simulink model "VoltageSourceConverterHVDCTrans"  (R2025b)
settings: Solver=FixedStepDiscrete  StartTime=0.0  StopTime=5  FixedStep=Ts  MaxStep=1e-4  RelTol=1e-3
PreLoadFcn:
  | VoltageSourceConverterHVDCTransParameters
values from neighbouring files (symbols this model uses):
  c = 0.207e-6    (= 2.07e-07)    [VoltageSourceConverterHVDCTransParameters.m]
  Cf = ((QRatedFilter/(VRated^2*(2*pi*FRated)))*(n^2-1)/(n^2))/Cbase    [VoltageSourceConverterHVDCTransParameters.m]
  FRated = 60    [VoltageSourceConverterHVDCTransParameters.m]
  Idcbase = Pbase/VdcRated    (= 1000)    [VoltageSourceConverterHVDCTransParameters.m]
  IL0 = opIdc.get("I").Value.value    [VoltageSourceConverterHVDCTransInitializeModel.m]
  l = 0.189e-3    (= 0.000189)    [VoltageSourceConverterHVDCTransParameters.m]
  Lbase = Zbase/wbase    [VoltageSourceConverterHVDCTransParameters.m]
  Lr = 0.15    [VoltageSourceConverterHVDCTransParameters.m]
  n = 25    [VoltageSourceConverterHVDCTransParameters.m]
  PRated = 300e6    (= 300000000)    [VoltageSourceConverterHVDCTransParameters.m]
  r = 0.0376    [VoltageSourceConverterHVDCTransParameters.m]
  Rc = r*Dis    (= 11.28)    [VoltageSourceConverterHVDCTransParameters.m]
  Rr = 0.002    [VoltageSourceConverterHVDCTransParameters.m]
  Rt = 0.002625    [VoltageSourceConverterHVDCTransParameters.m]
  Ts = 1/(fsw*100)    [VoltageSourceConverterHVDCTransInitializeModel.m]    (also in VoltageSourceConverterHVDCTransParameters.m = 6.66666666667e-05; VoltageSourceConverterHVDCTransVariantControl.m)
  Tsc = 10*Ts    (= 0.166666666667)    [VoltageSourceConverterHVDCTransInitializeModel.m]    (also in VoltageSourceConverterHVDCTransParameters.m = 6.66666666667e-05; VoltageSourceConverterHVDCTransVariantControl.m)
  Vdcr0 = 2*opReceivingEndVdcp.get("V").Value.value    [VoltageSourceConverterHVDCTransInitializeModel.m]
  VdcRated = 300e3    (= 300000)    [VoltageSourceConverterHVDCTransParameters.m]
  Vdcs0 = 2*opSendingEndVdcp.get("V").Value.value    [VoltageSourceConverterHVDCTransInitializeModel.m]
  VRated = 150e3    (= 150000)    [VoltageSourceConverterHVDCTransParameters.m]
  Xt = 0.19197    [VoltageSourceConverterHVDCTransParameters.m]
  Zbase = Vbase/Ibase    [VoltageSourceConverterHVDCTransParameters.m]
undefined symbols (not defined in the file or in its folder): DiscIntNeverNeededParam
libraries: nesl_utility x43, fl_lib x32, ee_lib x22, eeTransforms x16, eeGeneralControl x14, slpidlib x13, mcbeeMathTransformLib x8, eeSinusoidalMeasurement x2, eePwmGeneratorThreeLevel x2
(part 4 of 4)

== system VoltageSourceConverterHVDCTrans/Control/Sending end and receiving end control/Receiving end control/Time mode/Receiving-end Control/DC voltage and reactive power control ==
  VdcRef : Inport
  Vdcp : Inport  Port=2
  Vdcn : Inport  Port=3
  Qref : Inport  Port=4
  Qmea : Inport  Port=5
  Add2 : Sum
  Gain : Gain  Gain=-1
  Gain1 : Gain  Gain=VdcRated/Vbase
  Gain2 : Gain  Gain=0.5
  P PI : slpidlib/PID Controller  Controller=PI  Form=Parallel  TimeDomain=Discrete-time  UseExternalTs=off  SampleTime=Tsc  IntegratorMethod=Forward Euler  FilterMethod=Forward Euler  ControllerParametersSource=internal  P=REnd_Vdc_PI(1)  I=REnd_Vdc_PI(2)  UseKiTs=off  D=0  UseExternalDerivativeSource=off  N=100  UseFilter=on  TunerSelectOption=Transfer Function Based (PID Tuner App)  InitialConditionSource=internal  InitialConditionForIntegrator=P_PIr0  InitialConditionForFilter=0  DifferentiatorICPrevScaledInput=0  ExternalReset=none  TrackingMode=off  Kt=1  LimitOutput=on  SatLimitsSource=internal  UpperSaturationLimit=1.5  LowerSaturationLimit=-1.5  LinearizeAsGain=on  AntiWindupMode=back-calculation  Kb=1000  LimitIntegrator=off  UpperIntegratorSaturationLimit=1.2  LowerIntegratorSaturationLimit=-1.2  POutMin=[]  POutMax=[]  IOutMin=[]  IOutMax=[]  DOutMin=[]  DOutMax=[]  NOutMin=[]  NOutMax=[]  SumOutMin=[]  SumOutMax=[]  SaturationOutMin=[]  SaturationOutMax=[]  PParamMin=[]  PParamMax=[]  IParamMin=[]  IParamMax=[]  DParamMin=[]  DParamMax=[]  NParamMin=[]  NParamMax=[]  KbParamMin=[]  KbParamMax=[]  KtParamMin=[]  KtParamMax=[]  KbOutMin=[]  KbOutMax=[]  KtOutMin=[]  KtOutMax=[]  IntegratorOutMin=[]  IntegratorOutMax=[]  FilterOutMin=[]  FilterOutMax=[]  SumI1OutMin=[]  SumI1OutMax=[]  SumI2OutMin=[]  SumI2OutMax=[]  SumI3OutMin=[]  SumI3OutMax=[]  SumI4OutMin=[]  SumI4OutMax=[]  SumDOutMin=[]  SumDOutMax=[]  DifferentiatorOutMin=[]  DifferentiatorOutMax=[]  FilterDiffOutCoefMin=[]  FilterDiffOutCoefMax=[]  ReciprocalOutMin=[]  ReciprocalOutMax=[]  SumDenOutMin=[]  SumDenOutMax=[]  SumNumOutMin=[]  SumNumOutMax=[]  DivideOutMin=[]  DivideOutMax=[]  UdiffTsProdOutMin=[]  UdiffTsProdOutMax=[]  NTsProdOutMin=[]  NTsProdOutMax=[]  UintegralTsProdOutMin=[]  UintegralTsProdOutMax=[]  UngainTsProdOutMin=[]  UngainTsProdOutMax=[]  ClampingZeroOutDataTypeStr=Inherit: Inherit via back propagation  ClampingZeroOutMin=[]  ClampingZeroOutMax=[]  FilterDenConstantOutDataTypeStr=Inherit: Inherit via back propagation  FilterDenConstantOutMin=[]  FilterDenConstantOutMax=[]  PCopyOutDataTypeStr=Inherit: Inherit via back propagation  PCopyOutMin=[]  PCopyOutMax=[]  NCopyOutDataTypeStr=Inherit: Inherit via back propagation  NCopyOutMin=[]  NCopyOutMax=[]  IntegratorContinuousStateAttributes=''  IntegratorStateMustResolveToSignalObject=off  IntegratorRTWStateStorageClass=Auto  FilterContinuousStateAttributes=''  FilterStateMustResolveToSignalObject=off  FilterRTWStateStorageClass=Auto  ParallelPVariant=InternalParameters  IdealPVariant=Disabled  IVariant=InternalParameters  DVariant=Disabled  IntegratorVariant=Discrete  SatVariant=Enabled  AWVariant=BackCalculation  PCopyVariant=Disabled  TRVariant=Disabled  FdbkBlocksVariant=Forward  IdealPFdbkVariant=Disabled  SatFdbkVariant=Disabled  DerivativeFilterVariant=Disabled  NVariant=Disabled  NCopyVariant=Disabled_SignalSpec  FilterICVariant=Disabled  IntegratorICVariant=InternalICs  ExternalResetVariant=Disabled  TRSumVariant=Passthrough  SumFdbkVariant=Disabled  SumVariant=Sum_PI  TsampFilterVariant=InternalTs  TsampNgainVariant=Passthrough  TsampIntegralVariant=Disabled_SignalSpec  ExternalSaturationOutDataTypeStr=Inherit: Same as second input  DerivativeSourceVariant=Disabled  PreIntVariant=InternalPreInt
  Q PI : slpidlib/PID Controller  Controller=PI  Form=Parallel  TimeDomain=Discrete-time  UseExternalTs=off  SampleTime=Tsc  IntegratorMethod=Forward Euler  FilterMethod=Forward Euler  ControllerParametersSource=internal  P=REnd_Q_PI(1)  I=REnd_Q_PI(2)  UseKiTs=off  D=0  UseExternalDerivativeSource=off  N=100  UseFilter=on  TunerSelectOption=Transfer Function Based (PID Tuner App)  InitialConditionSource=internal  InitialConditionForIntegrator=-Q_PIr0  InitialConditionForFilter=0  DifferentiatorICPrevScaledInput=0  ExternalReset=none  TrackingMode=off  Kt=1  LimitOutput=on  SatLimitsSource=internal  UpperSaturationLimit=1.5  LowerSaturationLimit=-1.5  LinearizeAsGain=on  AntiWindupMode=back-calculation  Kb=1000  LimitIntegrator=off  UpperIntegratorSaturationLimit=1.3  LowerIntegratorSaturationLimit=-1.3  POutMin=[]  POutMax=[]  IOutMin=[]  IOutMax=[]  DOutMin=[]  DOutMax=[]  NOutMin=[]  NOutMax=[]  SumOutMin=[]  SumOutMax=[]  SaturationOutMin=[]  SaturationOutMax=[]  PParamMin=[]  PParamMax=[]  IParamMin=[]  IParamMax=[]  DParamMin=[]  DParamMax=[]  NParamMin=[]  NParamMax=[]  KbParamMin=[]  KbParamMax=[]  KtParamMin=[]  KtParamMax=[]  KbOutMin=[]  KbOutMax=[]  KtOutMin=[]  KtOutMax=[]  IntegratorOutMin=[]  IntegratorOutMax=[]  FilterOutMin=[]  FilterOutMax=[]  SumI1OutMin=[]  SumI1OutMax=[]  SumI2OutMin=[]  SumI2OutMax=[]  SumI3OutMin=[]  SumI3OutMax=[]  SumI4OutMin=[]  SumI4OutMax=[]  SumDOutMin=[]  SumDOutMax=[]  DifferentiatorOutMin=[]  DifferentiatorOutMax=[]  FilterDiffOutCoefMin=[]  FilterDiffOutCoefMax=[]  ReciprocalOutMin=[]  ReciprocalOutMax=[]  SumDenOutMin=[]  SumDenOutMax=[]  SumNumOutMin=[]  SumNumOutMax=[]  DivideOutMin=[]  DivideOutMax=[]  UdiffTsProdOutMin=[]  UdiffTsProdOutMax=[]  NTsProdOutMin=[]  NTsProdOutMax=[]  UintegralTsProdOutMin=[]  UintegralTsProdOutMax=[]  UngainTsProdOutMin=[]  UngainTsProdOutMax=[]  ClampingZeroOutDataTypeStr=Inherit: Inherit via back propagation  ClampingZeroOutMin=[]  ClampingZeroOutMax=[]  FilterDenConstantOutDataTypeStr=Inherit: Inherit via back propagation  FilterDenConstantOutMin=[]  FilterDenConstantOutMax=[]  PCopyOutDataTypeStr=Inherit: Inherit via back propagation  PCopyOutMin=[]  PCopyOutMax=[]  NCopyOutDataTypeStr=Inherit: Inherit via back propagation  NCopyOutMin=[]  NCopyOutMax=[]  IntegratorContinuousStateAttributes=''  IntegratorStateMustResolveToSignalObject=off  IntegratorRTWStateStorageClass=Auto  FilterContinuousStateAttributes=''  FilterStateMustResolveToSignalObject=off  FilterRTWStateStorageClass=Auto  ParallelPVariant=InternalParameters  IdealPVariant=Disabled  IVariant=InternalParameters  DVariant=Disabled  IntegratorVariant=Discrete  SatVariant=Enabled  AWVariant=BackCalculation  PCopyVariant=Disabled  TRVariant=Disabled  FdbkBlocksVariant=Forward  IdealPFdbkVariant=Disabled  SatFdbkVariant=Disabled  DerivativeFilterVariant=Disabled  NVariant=Disabled  NCopyVariant=Disabled_SignalSpec  FilterICVariant=Disabled  IntegratorICVariant=InternalICs  ExternalResetVariant=Disabled  TRSumVariant=Passthrough  SumFdbkVariant=Disabled  SumVariant=Sum_PI  TsampFilterVariant=InternalTs  TsampNgainVariant=Passthrough  TsampIntegralVariant=Disabled_SignalSpec  ExternalSaturationOutDataTypeStr=Inherit: Same as second input  DerivativeSourceVariant=Disabled  PreIntVariant=InternalPreInt
  Sum5 : Sum  Inputs=|+-
  Sum6 : Sum  Inputs=|+-
  idRef : Outport
  iqRef : Outport  Port=2
  wires:
  Gain1/1 -> P PI/1
  Gain2/1 -> Sum5/2
  Vdcn/1 -> Add2/2
  Vdcp/1 -> Add2/1
  Add2/1 -> Gain2/1
  Gain/1 -> iqRef/1
  VdcRef/1 -> Sum5/1
  Qmea/1 -> Sum6/2
  Qref/1 -> Sum6/1
  Q PI/1 -> Gain/1
  Sum6/1 -> Q PI/1
  P PI/1 -> idRef/1
  Sum5/1 -> Gain1/1

== system VoltageSourceConverterHVDCTrans/Control/Sending end and receiving end control/Sending end control/Frequency-and-time mode/Control/Active and reactive power control ==
  Pref : Inport
  Pmea : Inport  Port=2
  Qref : Inport  Port=3
  Qmea : Inport  Port=4
  Gain : Gain  Gain=-1
  P PI : slpidlib/PID Controller  Controller=PI  Form=Parallel  TimeDomain=Discrete-time  UseExternalTs=off  SampleTime=Tsc  IntegratorMethod=Forward Euler  FilterMethod=Forward Euler  ControllerParametersSource=internal  P=SEnd_P_PI_Low(1)  I=SEnd_P_PI_Low(2)  UseKiTs=off  D=0  UseExternalDerivativeSource=off  N=100  UseFilter=on  TunerSelectOption=Transfer Function Based (PID Tuner App)  InitialConditionSource=internal  InitialConditionForIntegrator=P_PIs0  InitialConditionForFilter=0  DifferentiatorICPrevScaledInput=0  ExternalReset=none  TrackingMode=off  Kt=1  LimitOutput=on  SatLimitsSource=internal  UpperSaturationLimit=1.5  LowerSaturationLimit=-1.5  LinearizeAsGain=on  AntiWindupMode=back-calculation  Kb=1000  LimitIntegrator=off  UpperIntegratorSaturationLimit=inf  LowerIntegratorSaturationLimit=-inf  POutMin=[]  POutMax=[]  IOutMin=[]  IOutMax=[]  DOutMin=[]  DOutMax=[]  NOutMin=[]  NOutMax=[]  SumOutMin=[]  SumOutMax=[]  SaturationOutMin=[]  SaturationOutMax=[]  PParamMin=[]  PParamMax=[]  IParamMin=[]  IParamMax=[]  DParamMin=[]  DParamMax=[]  NParamMin=[]  NParamMax=[]  KbParamMin=[]  KbParamMax=[]  KtParamMin=[]  KtParamMax=[]  KbOutMin=[]  KbOutMax=[]  KtOutMin=[]  KtOutMax=[]  IntegratorOutMin=[]  IntegratorOutMax=[]  FilterOutMin=[]  FilterOutMax=[]  SumI1OutMin=[]  SumI1OutMax=[]  SumI2OutMin=[]  SumI2OutMax=[]  SumI3OutMin=[]  SumI3OutMax=[]  SumI4OutMin=[]  SumI4OutMax=[]  SumDOutMin=[]  SumDOutMax=[]  DifferentiatorOutMin=[]  DifferentiatorOutMax=[]  FilterDiffOutCoefMin=[]  FilterDiffOutCoefMax=[]  ReciprocalOutMin=[]  ReciprocalOutMax=[]  SumDenOutMin=[]  SumDenOutMax=[]  SumNumOutMin=[]  SumNumOutMax=[]  DivideOutMin=[]  DivideOutMax=[]  UdiffTsProdOutMin=[]  UdiffTsProdOutMax=[]  NTsProdOutMin=[]  NTsProdOutMax=[]  UintegralTsProdOutMin=[]  UintegralTsProdOutMax=[]  UngainTsProdOutMin=[]  UngainTsProdOutMax=[]  ClampingZeroOutDataTypeStr=Inherit: Inherit via back propagation  ClampingZeroOutMin=[]  ClampingZeroOutMax=[]  FilterDenConstantOutDataTypeStr=Inherit: Inherit via back propagation  FilterDenConstantOutMin=[]  FilterDenConstantOutMax=[]  PCopyOutDataTypeStr=Inherit: Inherit via back propagation  PCopyOutMin=[]  PCopyOutMax=[]  NCopyOutDataTypeStr=Inherit: Inherit via back propagation  NCopyOutMin=[]  NCopyOutMax=[]  IntegratorContinuousStateAttributes=''  IntegratorStateMustResolveToSignalObject=off  IntegratorRTWStateStorageClass=Auto  FilterContinuousStateAttributes=''  FilterStateMustResolveToSignalObject=off  FilterRTWStateStorageClass=Auto  ParallelPVariant=InternalParameters  IdealPVariant=Disabled  IVariant=InternalParameters  DVariant=Disabled  IntegratorVariant=Discrete  SatVariant=Enabled  AWVariant=BackCalculation  PCopyVariant=Disabled  TRVariant=Disabled  FdbkBlocksVariant=Forward  IdealPFdbkVariant=Disabled  SatFdbkVariant=Disabled  DerivativeFilterVariant=Disabled  NVariant=Disabled  NCopyVariant=Disabled_SignalSpec  FilterICVariant=Disabled  IntegratorICVariant=InternalICs  ExternalResetVariant=Disabled  TRSumVariant=Passthrough  SumFdbkVariant=Disabled  SumVariant=Sum_PI  TsampFilterVariant=InternalTs  TsampNgainVariant=Passthrough  TsampIntegralVariant=Disabled_SignalSpec  ExternalSaturationOutDataTypeStr=Inherit: Same as second input  DerivativeSourceVariant=Disabled  PreIntVariant=InternalPreInt
  Q PI : slpidlib/PID Controller  Controller=PI  Form=Parallel  TimeDomain=Discrete-time  UseExternalTs=off  SampleTime=Tsc  IntegratorMethod=Forward Euler  FilterMethod=Forward Euler  ControllerParametersSource=internal  P=SEnd_Q_PI_Low(1)  I=SEnd_Q_PI_Low(2)  UseKiTs=off  D=0  UseExternalDerivativeSource=off  N=100  UseFilter=on  TunerSelectOption=Transfer Function Based (PID Tuner App)  InitialConditionSource=internal  InitialConditionForIntegrator=-Q_PIs0  InitialConditionForFilter=0  DifferentiatorICPrevScaledInput=0  ExternalReset=none  TrackingMode=off  Kt=1  LimitOutput=on  SatLimitsSource=internal  UpperSaturationLimit=1.5  LowerSaturationLimit=-1.5  LinearizeAsGain=on  AntiWindupMode=back-calculation  Kb=1000  LimitIntegrator=off  UpperIntegratorSaturationLimit=inf  LowerIntegratorSaturationLimit=-inf  POutMin=[]  POutMax=[]  IOutMin=[]  IOutMax=[]  DOutMin=[]  DOutMax=[]  NOutMin=[]  NOutMax=[]  SumOutMin=[]  SumOutMax=[]  SaturationOutMin=[]  SaturationOutMax=[]  PParamMin=[]  PParamMax=[]  IParamMin=[]  IParamMax=[]  DParamMin=[]  DParamMax=[]  NParamMin=[]  NParamMax=[]  KbParamMin=[]  KbParamMax=[]  KtParamMin=[]  KtParamMax=[]  KbOutMin=[]  KbOutMax=[]  KtOutMin=[]  KtOutMax=[]  IntegratorOutMin=[]  IntegratorOutMax=[]  FilterOutMin=[]  FilterOutMax=[]  SumI1OutMin=[]  SumI1OutMax=[]  SumI2OutMin=[]  SumI2OutMax=[]  SumI3OutMin=[]  SumI3OutMax=[]  SumI4OutMin=[]  SumI4OutMax=[]  SumDOutMin=[]  SumDOutMax=[]  DifferentiatorOutMin=[]  DifferentiatorOutMax=[]  FilterDiffOutCoefMin=[]  FilterDiffOutCoefMax=[]  ReciprocalOutMin=[]  ReciprocalOutMax=[]  SumDenOutMin=[]  SumDenOutMax=[]  SumNumOutMin=[]  SumNumOutMax=[]  DivideOutMin=[]  DivideOutMax=[]  UdiffTsProdOutMin=[]  UdiffTsProdOutMax=[]  NTsProdOutMin=[]  NTsProdOutMax=[]  UintegralTsProdOutMin=[]  UintegralTsProdOutMax=[]  UngainTsProdOutMin=[]  UngainTsProdOutMax=[]  ClampingZeroOutDataTypeStr=Inherit: Inherit via back propagation  ClampingZeroOutMin=[]  ClampingZeroOutMax=[]  FilterDenConstantOutDataTypeStr=Inherit: Inherit via back propagation  FilterDenConstantOutMin=[]  FilterDenConstantOutMax=[]  PCopyOutDataTypeStr=Inherit: Inherit via back propagation  PCopyOutMin=[]  PCopyOutMax=[]  NCopyOutDataTypeStr=Inherit: Inherit via back propagation  NCopyOutMin=[]  NCopyOutMax=[]  IntegratorContinuousStateAttributes=''  IntegratorStateMustResolveToSignalObject=off  IntegratorRTWStateStorageClass=Auto  FilterContinuousStateAttributes=''  FilterStateMustResolveToSignalObject=off  FilterRTWStateStorageClass=Auto  ParallelPVariant=InternalParameters  IdealPVariant=Disabled  IVariant=InternalParameters  DVariant=Disabled  IntegratorVariant=Discrete  SatVariant=Enabled  AWVariant=BackCalculation  PCopyVariant=Disabled  TRVariant=Disabled  FdbkBlocksVariant=Forward  IdealPFdbkVariant=Disabled  SatFdbkVariant=Disabled  DerivativeFilterVariant=Disabled  NVariant=Disabled  NCopyVariant=Disabled_SignalSpec  FilterICVariant=Disabled  IntegratorICVariant=InternalICs  ExternalResetVariant=Disabled  TRSumVariant=Passthrough  SumFdbkVariant=Disabled  SumVariant=Sum_PI  TsampFilterVariant=InternalTs  TsampNgainVariant=Passthrough  TsampIntegralVariant=Disabled_SignalSpec  ExternalSaturationOutDataTypeStr=Inherit: Same as second input  DerivativeSourceVariant=Disabled  PreIntVariant=InternalPreInt
  Sum5 : Sum  Inputs=|+-
  Sum6 : Sum  Inputs=|+-
  idRef : Outport
  iqRef : Outport  Port=2
  wires:
  Pmea/1 -> Sum5/2
  Gain/1 -> iqRef/1
  Pref/1 -> Sum5/1
  Qmea/1 -> Sum6/2
  Qref/1 -> Sum6/1
  Q PI/1 -> Gain/1
  Sum6/1 -> Q PI/1
  P PI/1 -> idRef/1
  Sum5/1 -> P PI/1

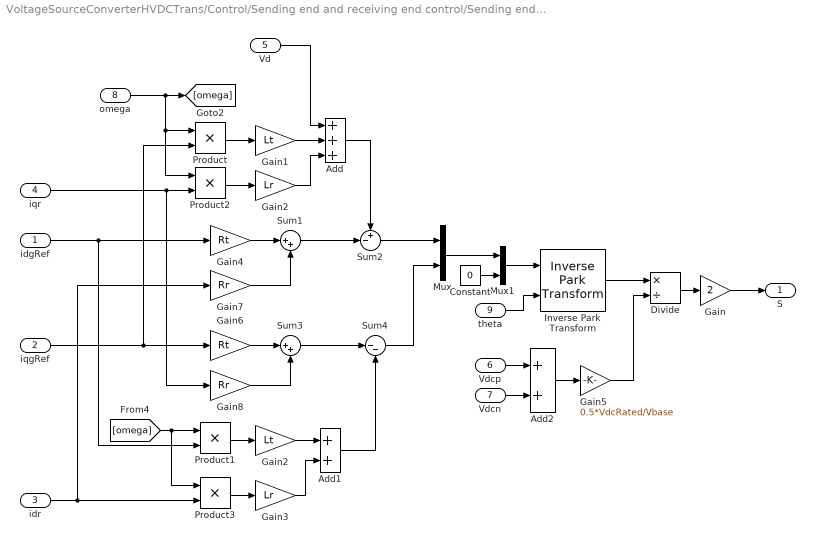
== system VoltageSourceConverterHVDCTrans/Control/Sending end and receiving end control/Sending end control/Frequency-and-time mode/Control/Current control ==
  idgRef : Inport
  iqgRef : Inport  Port=2
  idr : Inport  Port=3
  iqr : Inport  Port=4
  Vd : Inport  Port=5
  Vdcp : Inport  Port=6
  Vdcn : Inport  Port=7
  omega : Inport  Port=8
  theta : Inport  Port=9
  Add : Sum  Inputs=+++
  Add1 : Sum
  Add2 : Sum
  Constant : Constant  Value=0  SampleTime=Tsc
  Divide : Product  Inputs=*/
  Gain : Gain  Gain=2
  Gain1 : Gain  Gain=Lt
  Gain2 : Gain  Gain=Lr
  "Gain2 " : Gain  Gain=Lt
  Gain3 : Gain  Gain=Lr
  Gain4 : Gain  Gain=Rt
  Gain5 : Gain  Gain=0.5*VdcRated/Vbase
  Gain6 : Gain  Gain=Rt
  Gain7 : Gain  Gain=Rr
  Gain8 : Gain  Gain=Rr
  Inverse Park Transform : eeTransforms/Inverse Park Transform  AxisAlignment=Q-axis  PowerInvariant=off
  Mux : Mux  Inputs=2
  Mux1 : Mux  Inputs=2
  Product{,1..3} (4 alike) : Product  Inputs=**
  Sum1 : Sum  Inputs=|++
  Sum2 : Sum  Inputs=+-|
  Sum3 : Sum  Inputs=|++
  Sum4 : Sum  Inputs=|--
  S : Outport
  wires:
  Vd/1 -> Add/1
  Mux/1 -> Mux1/1
  idgRef/1 -> Product1/2, Gain4/1
  Constant/1 -> Mux1/2
  Inverse Park Transform/1 -> Divide/1
  Mux1/1 -> Inverse Park Transform/1
  iqgRef/1 -> Product/2, Gain6/1
  omega/1 -> Product2/1, Product/1, [omega]
  [omega] -> Product3/1, Product1/1
  Product/1 -> Gain1/1
  Sum4/1 -> Mux/2
  Product1/1 -> "Gain2 "/1
  Add/1 -> Sum2/1
  theta/1 -> Inverse Park Transform/2
  Gain1/1 -> Add/2
  Sum2/1 -> Mux/1
  iqr/1 -> Product2/2, Gain8/1
  Product2/1 -> Gain2/1
  Gain2/1 -> Add/3
  idr/1 -> Gain7/1, Product3/2
  Product3/1 -> Gain3/1
  "Gain2 "/1 -> Add1/1
  Gain3/1 -> Add1/2
  Add1/1 -> Sum4/2
  Divide/1 -> Gain/1
  Sum1/1 -> Sum2/2
  Sum3/1 -> Sum4/1
  Add2/1 -> Gain5/1
  Gain5/1 -> Divide/2
  Gain/1 -> S/1
  Gain4/1 -> Sum1/1
  Gain7/1 -> Sum1/2
  Gain6/1 -> Sum3/1
  Gain8/1 -> Sum3/2
  Vdcp/1 -> Add2/1
  Vdcn/1 -> Add2/2

== system VoltageSourceConverterHVDCTrans/Control/Sending end and receiving end control/Sending end control/Frequency-and-time mode/Measurements/Clarke ==
  abc : Inport
  0 : Fcn  Expr=u(1) + u(2) + u(3)
  K : Gain  Gain=[2 2 1]/3
  Mux : Mux  Inputs=3
  alpha : Fcn  Expr=(u(1) - u(3))*sqrt(3)/2
  beta : Fcn  Expr=-0.5*u(1) + u(2) -0.5*u(3)
  AlphaBeta0 : Outport
  wires:
  beta/1 -> Mux/2
  Mux/1 -> K/1
  abc/1 -> alpha/1, beta/1, 0/1
  alpha/1 -> Mux/1
  0/1 -> Mux/3
  K/1 -> AlphaBeta0/1

== system VoltageSourceConverterHVDCTrans/Control/Sending end and receiving end control/Sending end control/Frequency-and-time mode/Measurements/Clarke1 ==
  abc : Inport
  0 : Fcn  Expr=u(1) + u(2) + u(3)
  K : Gain  Gain=[2 2 1]/3
  Mux : Mux  Inputs=3
  alpha : Fcn  Expr=(u(1) - u(3))*sqrt(3)/2
  beta : Fcn  Expr=-0.5*u(1) + u(2) -0.5*u(3)
  AlphaBeta0 : Outport
  wires:
  K/1 -> AlphaBeta0/1
  0/1 -> Mux/3
  alpha/1 -> Mux/1
  abc/1 -> 0/1, beta/1, alpha/1
  Mux/1 -> K/1
  beta/1 -> Mux/2

== system VoltageSourceConverterHVDCTrans/Control/Sending end and receiving end control/Sending end control/Frequency-and-time mode/Measurements/PQ Calculation ==
  Vd : Inport
  Id : Inport  Port=2
  Iq : Inport  Port=3
  Gain : Gain  Gain=-1
  Product : Product
  Product4 : Product
  P : Outport
  Q : Outport  Port=2
  wires:
  Vd/1 -> Product4/1, Product/1
  Product/1 -> P/1
  Id/1 -> Product/2
  Iq/1 -> Product4/2
  Product4/1 -> Gain/1
  Gain/1 -> Q/1

== system VoltageSourceConverterHVDCTrans/Control/Sending end and receiving end control/Sending end control/Frequency-and-time mode/Measurements/Phase calculation ==
  Vabcg : Inport
  Divide : Product  Inputs=*/
  Gain : Gain  Gain=2/3
  Math Function : Math  Operator=square
  Selector : Selector  InputPortWidth=3  IndexOptions=Index vector (dialog)  Indices=[1]  OutputSizes=1
  Sqrt : Sqrt
  Sum of Elements : Sum  Inputs=+
  Trigonometric Function : Trigonometry  Operator=asin
  Phase : Outport
  wires:
  Sqrt/1 -> Divide/2
  Divide/1 -> Trigonometric Function/1
  Vabcg/1 -> Selector/1, Math Function/1
  Gain/1 -> Sqrt/1
  Selector/1 -> Divide/1
  Sum of Elements/1 -> Gain/1
  Math Function/1 -> Sum of Elements/1
  Trigonometric Function/1 -> Phase/1

== system VoltageSourceConverterHVDCTrans/Control/Sending end and receiving end control/Sending end control/Time mode/Control/Active and reactive power control ==
  Pref : Inport
  Pmea : Inport  Port=2
  Qref : Inport  Port=3
  Qmea : Inport  Port=4
  Gain : Gain  Gain=-1
  P PI : slpidlib/PID Controller  Controller=PI  Form=Parallel  TimeDomain=Discrete-time  UseExternalTs=off  SampleTime=Tsc  IntegratorMethod=Forward Euler  FilterMethod=Forward Euler  ControllerParametersSource=internal  P=SEnd_P_PI(1)  I=SEnd_P_PI(2)  UseKiTs=off  D=0  UseExternalDerivativeSource=off  N=100  UseFilter=on  TunerSelectOption=Transfer Function Based (PID Tuner App)  InitialConditionSource=internal  InitialConditionForIntegrator=P_PIs0  InitialConditionForFilter=0  DifferentiatorICPrevScaledInput=0  ExternalReset=none  TrackingMode=off  Kt=1  LimitOutput=on  SatLimitsSource=internal  UpperSaturationLimit=1.5  LowerSaturationLimit=-1.5  LinearizeAsGain=on  AntiWindupMode=back-calculation  Kb=1000  LimitIntegrator=off  UpperIntegratorSaturationLimit=1.2  LowerIntegratorSaturationLimit=-1.2  POutMin=[]  POutMax=[]  IOutMin=[]  IOutMax=[]  DOutMin=[]  DOutMax=[]  NOutMin=[]  NOutMax=[]  SumOutMin=[]  SumOutMax=[]  SaturationOutMin=[]  SaturationOutMax=[]  PParamMin=[]  PParamMax=[]  IParamMin=[]  IParamMax=[]  DParamMin=[]  DParamMax=[]  NParamMin=[]  NParamMax=[]  KbParamMin=[]  KbParamMax=[]  KtParamMin=[]  KtParamMax=[]  KbOutMin=[]  KbOutMax=[]  KtOutMin=[]  KtOutMax=[]  IntegratorOutMin=[]  IntegratorOutMax=[]  FilterOutMin=[]  FilterOutMax=[]  SumI1OutMin=[]  SumI1OutMax=[]  SumI2OutMin=[]  SumI2OutMax=[]  SumI3OutMin=[]  SumI3OutMax=[]  SumI4OutMin=[]  SumI4OutMax=[]  SumDOutMin=[]  SumDOutMax=[]  DifferentiatorOutMin=[]  DifferentiatorOutMax=[]  FilterDiffOutCoefMin=[]  FilterDiffOutCoefMax=[]  ReciprocalOutMin=[]  ReciprocalOutMax=[]  SumDenOutMin=[]  SumDenOutMax=[]  SumNumOutMin=[]  SumNumOutMax=[]  DivideOutMin=[]  DivideOutMax=[]  UdiffTsProdOutMin=[]  UdiffTsProdOutMax=[]  NTsProdOutMin=[]  NTsProdOutMax=[]  UintegralTsProdOutMin=[]  UintegralTsProdOutMax=[]  UngainTsProdOutMin=[]  UngainTsProdOutMax=[]  ClampingZeroOutDataTypeStr=Inherit: Inherit via back propagation  ClampingZeroOutMin=[]  ClampingZeroOutMax=[]  FilterDenConstantOutDataTypeStr=Inherit: Inherit via back propagation  FilterDenConstantOutMin=[]  FilterDenConstantOutMax=[]  PCopyOutDataTypeStr=Inherit: Inherit via back propagation  PCopyOutMin=[]  PCopyOutMax=[]  NCopyOutDataTypeStr=Inherit: Inherit via back propagation  NCopyOutMin=[]  NCopyOutMax=[]  IntegratorContinuousStateAttributes=''  IntegratorStateMustResolveToSignalObject=off  IntegratorRTWStateStorageClass=Auto  FilterContinuousStateAttributes=''  FilterStateMustResolveToSignalObject=off  FilterRTWStateStorageClass=Auto  ParallelPVariant=InternalParameters  IdealPVariant=Disabled  IVariant=InternalParameters  DVariant=Disabled  IntegratorVariant=Discrete  SatVariant=Enabled  AWVariant=BackCalculation  PCopyVariant=Disabled  TRVariant=Disabled  FdbkBlocksVariant=Forward  IdealPFdbkVariant=Disabled  SatFdbkVariant=Disabled  DerivativeFilterVariant=Disabled  NVariant=Disabled  NCopyVariant=Disabled_SignalSpec  FilterICVariant=Disabled  IntegratorICVariant=InternalICs  ExternalResetVariant=Disabled  TRSumVariant=Passthrough  SumFdbkVariant=Disabled  SumVariant=Sum_PI  TsampFilterVariant=InternalTs  TsampNgainVariant=Passthrough  TsampIntegralVariant=Disabled_SignalSpec  ExternalSaturationOutDataTypeStr=Inherit: Same as second input  DerivativeSourceVariant=Disabled  PreIntVariant=InternalPreInt
  Q PI : slpidlib/PID Controller  Controller=PI  Form=Parallel  TimeDomain=Discrete-time  UseExternalTs=off  SampleTime=Tsc  IntegratorMethod=Forward Euler  FilterMethod=Forward Euler  ControllerParametersSource=internal  P=SEnd_Q_PI(1)  I=SEnd_Q_PI(2)  UseKiTs=off  D=0  UseExternalDerivativeSource=off  N=100  UseFilter=on  TunerSelectOption=Transfer Function Based (PID Tuner App)  InitialConditionSource=internal  InitialConditionForIntegrator=-Q_PIs0  InitialConditionForFilter=0  DifferentiatorICPrevScaledInput=0  ExternalReset=none  TrackingMode=off  Kt=1  LimitOutput=on  SatLimitsSource=internal  UpperSaturationLimit=1.5  LowerSaturationLimit=-1.5  LinearizeAsGain=on  AntiWindupMode=back-calculation  Kb=1000  LimitIntegrator=off  UpperIntegratorSaturationLimit=0.3  LowerIntegratorSaturationLimit=-0.3  POutMin=[]  POutMax=[]  IOutMin=[]  IOutMax=[]  DOutMin=[]  DOutMax=[]  NOutMin=[]  NOutMax=[]  SumOutMin=[]  SumOutMax=[]  SaturationOutMin=[]  SaturationOutMax=[]  PParamMin=[]  PParamMax=[]  IParamMin=[]  IParamMax=[]  DParamMin=[]  DParamMax=[]  NParamMin=[]  NParamMax=[]  KbParamMin=[]  KbParamMax=[]  KtParamMin=[]  KtParamMax=[]  KbOutMin=[]  KbOutMax=[]  KtOutMin=[]  KtOutMax=[]  IntegratorOutMin=[]  IntegratorOutMax=[]  FilterOutMin=[]  FilterOutMax=[]  SumI1OutMin=[]  SumI1OutMax=[]  SumI2OutMin=[]  SumI2OutMax=[]  SumI3OutMin=[]  SumI3OutMax=[]  SumI4OutMin=[]  SumI4OutMax=[]  SumDOutMin=[]  SumDOutMax=[]  DifferentiatorOutMin=[]  DifferentiatorOutMax=[]  FilterDiffOutCoefMin=[]  FilterDiffOutCoefMax=[]  ReciprocalOutMin=[]  ReciprocalOutMax=[]  SumDenOutMin=[]  SumDenOutMax=[]  SumNumOutMin=[]  SumNumOutMax=[]  DivideOutMin=[]  DivideOutMax=[]  UdiffTsProdOutMin=[]  UdiffTsProdOutMax=[]  NTsProdOutMin=[]  NTsProdOutMax=[]  UintegralTsProdOutMin=[]  UintegralTsProdOutMax=[]  UngainTsProdOutMin=[]  UngainTsProdOutMax=[]  ClampingZeroOutDataTypeStr=Inherit: Inherit via back propagation  ClampingZeroOutMin=[]  ClampingZeroOutMax=[]  FilterDenConstantOutDataTypeStr=Inherit: Inherit via back propagation  FilterDenConstantOutMin=[]  FilterDenConstantOutMax=[]  PCopyOutDataTypeStr=Inherit: Inherit via back propagation  PCopyOutMin=[]  PCopyOutMax=[]  NCopyOutDataTypeStr=Inherit: Inherit via back propagation  NCopyOutMin=[]  NCopyOutMax=[]  IntegratorContinuousStateAttributes=''  IntegratorStateMustResolveToSignalObject=off  IntegratorRTWStateStorageClass=Auto  FilterContinuousStateAttributes=''  FilterStateMustResolveToSignalObject=off  FilterRTWStateStorageClass=Auto  ParallelPVariant=InternalParameters  IdealPVariant=Disabled  IVariant=InternalParameters  DVariant=Disabled  IntegratorVariant=Discrete  SatVariant=Enabled  AWVariant=BackCalculation  PCopyVariant=Disabled  TRVariant=Disabled  FdbkBlocksVariant=Forward  IdealPFdbkVariant=Disabled  SatFdbkVariant=Disabled  DerivativeFilterVariant=Disabled  NVariant=Disabled  NCopyVariant=Disabled_SignalSpec  FilterICVariant=Disabled  IntegratorICVariant=InternalICs  ExternalResetVariant=Disabled  TRSumVariant=Passthrough  SumFdbkVariant=Disabled  SumVariant=Sum_PI  TsampFilterVariant=InternalTs  TsampNgainVariant=Passthrough  TsampIntegralVariant=Disabled_SignalSpec  ExternalSaturationOutDataTypeStr=Inherit: Same as second input  DerivativeSourceVariant=Disabled  PreIntVariant=InternalPreInt
  Sum5 : Sum  Inputs=|+-
  Sum6 : Sum  Inputs=|+-
  idRef : Outport
  iqRef : Outport  Port=2
  wires:
  Pmea/1 -> Sum5/2
  Gain/1 -> iqRef/1
  Pref/1 -> Sum5/1
  Qmea/1 -> Sum6/2
  Qref/1 -> Sum6/1
  Q PI/1 -> Gain/1
  Sum6/1 -> Q PI/1
  P PI/1 -> idRef/1
  Sum5/1 -> P PI/1

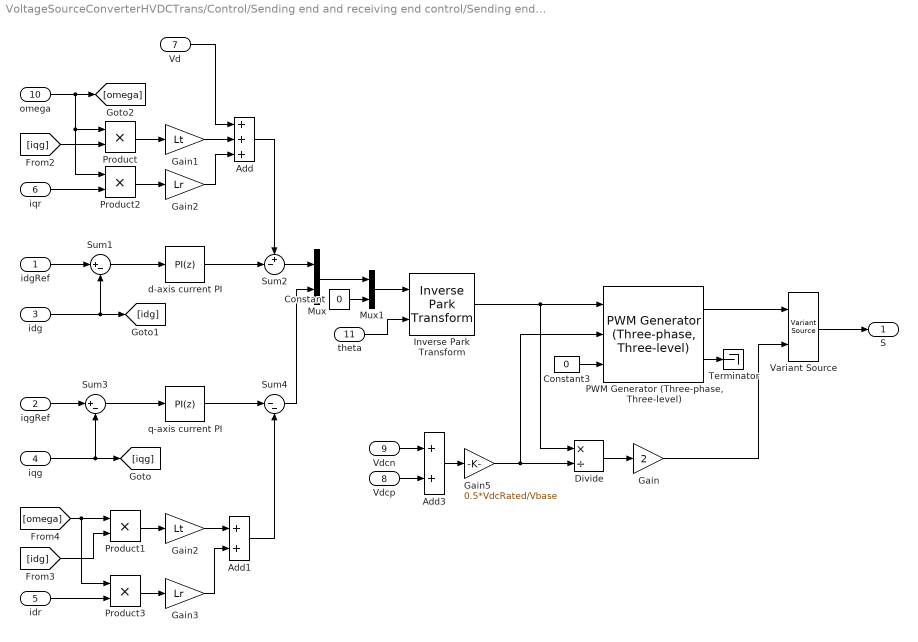
== system VoltageSourceConverterHVDCTrans/Control/Sending end and receiving end control/Sending end control/Time mode/Control/Current control ==
  idgRef : Inport
  iqgRef : Inport  Port=2
  idg : Inport  Port=3
  iqg : Inport  Port=4
  idr : Inport  Port=5
  iqr : Inport  Port=6
  Vd : Inport  Port=7
  Vdcp : Inport  Port=8
  Vdcn : Inport  Port=9
  omega : Inport  Port=10
  theta : Inport  Port=11
  Add : Sum  Inputs=+++
  Add1 : Sum
  Add3 : Sum
  Constant : Constant  Value=0  SampleTime=Tsc
  Constant3 : Constant  Value=0
  Divide : Product  Inputs=*/
  Gain : Gain  Gain=2
  Gain1 : Gain  Gain=Lt
  Gain2 : Gain  Gain=Lr
  "Gain2 " : Gain  Gain=Lt
  Gain3 : Gain  Gain=Lr
  Gain5 : Gain  Gain=0.5*VdcRated/Vbase
  Inverse Park Transform : eeTransforms/Inverse Park Transform  AxisAlignment=Q-axis  PowerInvariant=off
  Mux : Mux  Inputs=2
  Mux1 : Mux  Inputs=2
  "PWM Generator (Three-phase, Three-level)" : eePwmGeneratorThreeLevel/PWM Generator (Three-phase, Three-level)  CPWMMode=SPWM: sinusoidal PWM  fsw=fsw  Ts=Ts
      settings: SamplingMode=Natural
      settings: LibrarySourceBlock=|
      | ee_sl_lib/Pulse Width
      | Modulation/PWM Generator
      | (Three-phase, Three-level)
  Product{,1..3} (4 alike) : Product  Inputs=**
  Sum1 : Sum  Inputs=|+-
  Sum2 : Sum  Inputs=+-|
  Sum3 : Sum  Inputs=|+-
  Sum4 : Sum  Inputs=|--
  Terminator : Terminator
  Variant Source : VariantSource  ShowConditionOnBlock=on  VariantControls={SwitchingVSC, AverageValueVSC}
  d-axis current PI : slpidlib/PID Controller  Controller=PI  Form=Parallel  TimeDomain=Discrete-time  UseExternalTs=off  SampleTime=Tsc  IntegratorMethod=Forward Euler  FilterMethod=Forward Euler  ControllerParametersSource=internal  P=SEnd_Id_PI(1)  I=SEnd_Id_PI(2)  UseKiTs=off  D=0  UseExternalDerivativeSource=off  N=100  UseFilter=on  TunerSelectOption=Transfer Function Based (PID Tuner App)  InitialConditionSource=internal  InitialConditionForIntegrator=Id_PIs0  InitialConditionForFilter=0  DifferentiatorICPrevScaledInput=0  ExternalReset=none  TrackingMode=off  Kt=1  LimitOutput=on  SatLimitsSource=internal  UpperSaturationLimit=(Rt+Rr)*40  LowerSaturationLimit=-(Rt+Rr)*40  LinearizeAsGain=on  AntiWindupMode=back-calculation  Kb=1000  LimitIntegrator=off  UpperIntegratorSaturationLimit=inf  LowerIntegratorSaturationLimit=-inf  POutMin=[]  POutMax=[]  IOutMin=[]  IOutMax=[]  DOutMin=[]  DOutMax=[]  NOutMin=[]  NOutMax=[]  SumOutMin=[]  SumOutMax=[]  SaturationOutMin=[]  SaturationOutMax=[]  PParamMin=[]  PParamMax=[]  IParamMin=[]  IParamMax=[]  DParamMin=[]  DParamMax=[]  NParamMin=[]  NParamMax=[]  KbParamMin=[]  KbParamMax=[]  KtParamMin=[]  KtParamMax=[]  KbOutMin=[]  KbOutMax=[]  KtOutMin=[]  KtOutMax=[]  IntegratorOutMin=[]  IntegratorOutMax=[]  FilterOutMin=[]  FilterOutMax=[]  SumI1OutMin=[]  SumI1OutMax=[]  SumI2OutMin=[]  SumI2OutMax=[]  SumI3OutMin=[]  SumI3OutMax=[]  SumI4OutMin=[]  SumI4OutMax=[]  SumDOutMin=[]  SumDOutMax=[]  DifferentiatorOutMin=[]  DifferentiatorOutMax=[]  FilterDiffOutCoefMin=[]  FilterDiffOutCoefMax=[]  ReciprocalOutMin=[]  ReciprocalOutMax=[]  SumDenOutMin=[]  SumDenOutMax=[]  SumNumOutMin=[]  SumNumOutMax=[]  DivideOutMin=[]  DivideOutMax=[]  UdiffTsProdOutMin=[]  UdiffTsProdOutMax=[]  NTsProdOutMin=[]  NTsProdOutMax=[]  UintegralTsProdOutMin=[]  UintegralTsProdOutMax=[]  UngainTsProdOutMin=[]  UngainTsProdOutMax=[]  ClampingZeroOutDataTypeStr=Inherit: Inherit via back propagation  ClampingZeroOutMin=[]  ClampingZeroOutMax=[]  FilterDenConstantOutDataTypeStr=Inherit: Inherit via back propagation  FilterDenConstantOutMin=[]  FilterDenConstantOutMax=[]  PCopyOutDataTypeStr=Inherit: Inherit via back propagation  PCopyOutMin=[]  PCopyOutMax=[]  NCopyOutDataTypeStr=Inherit: Inherit via back propagation  NCopyOutMin=[]  NCopyOutMax=[]  IntegratorContinuousStateAttributes=''  IntegratorStateMustResolveToSignalObject=off  IntegratorRTWStateStorageClass=Auto  FilterContinuousStateAttributes=''  FilterStateMustResolveToSignalObject=off  FilterRTWStateStorageClass=Auto  ParallelPVariant=InternalParameters  IdealPVariant=Disabled  IVariant=InternalParameters  DVariant=Disabled  IntegratorVariant=Discrete  SatVariant=Enabled  AWVariant=BackCalculation  PCopyVariant=Disabled  TRVariant=Disabled  FdbkBlocksVariant=Forward  IdealPFdbkVariant=Disabled  SatFdbkVariant=Disabled  DerivativeFilterVariant=Disabled  NVariant=Disabled  NCopyVariant=Disabled_SignalSpec  FilterICVariant=Disabled  IntegratorICVariant=InternalICs  ExternalResetVariant=Disabled  TRSumVariant=Passthrough  SumFdbkVariant=Disabled  SumVariant=Sum_PI  TsampFilterVariant=InternalTs  TsampNgainVariant=Passthrough  TsampIntegralVariant=Disabled_SignalSpec  ExternalSaturationOutDataTypeStr=Inherit: Same as second input  DerivativeSourceVariant=Disabled  PreIntVariant=InternalPreInt
  q-axis current PI : slpidlib/PID Controller  Controller=PI  Form=Parallel  TimeDomain=Discrete-time  UseExternalTs=off  SampleTime=Tsc  IntegratorMethod=Forward Euler  FilterMethod=Forward Euler  ControllerParametersSource=internal  P=SEnd_Iq_PI(1)  I=SEnd_Iq_PI(2)  UseKiTs=off  D=0  UseExternalDerivativeSource=off  N=100  UseFilter=on  TunerSelectOption=Transfer Function Based (PID Tuner App)  InitialConditionSource=internal  InitialConditionForIntegrator=Iq_PIs0  InitialConditionForFilter=0  DifferentiatorICPrevScaledInput=0  ExternalReset=none  TrackingMode=off  Kt=1  LimitOutput=on  SatLimitsSource=internal  UpperSaturationLimit=(Rt+Rr)*40  LowerSaturationLimit=-(Rt+Rr)*40  LinearizeAsGain=on  AntiWindupMode=back-calculation  Kb=1000  LimitIntegrator=off  UpperIntegratorSaturationLimit=inf  LowerIntegratorSaturationLimit=-inf  POutMin=[]  POutMax=[]  IOutMin=[]  IOutMax=[]  DOutMin=[]  DOutMax=[]  NOutMin=[]  NOutMax=[]  SumOutMin=[]  SumOutMax=[]  SaturationOutMin=[]  SaturationOutMax=[]  PParamMin=[]  PParamMax=[]  IParamMin=[]  IParamMax=[]  DParamMin=[]  DParamMax=[]  NParamMin=[]  NParamMax=[]  KbParamMin=[]  KbParamMax=[]  KtParamMin=[]  KtParamMax=[]  KbOutMin=[]  KbOutMax=[]  KtOutMin=[]  KtOutMax=[]  IntegratorOutMin=[]  IntegratorOutMax=[]  FilterOutMin=[]  FilterOutMax=[]  SumI1OutMin=[]  SumI1OutMax=[]  SumI2OutMin=[]  SumI2OutMax=[]  SumI3OutMin=[]  SumI3OutMax=[]  SumI4OutMin=[]  SumI4OutMax=[]  SumDOutMin=[]  SumDOutMax=[]  DifferentiatorOutMin=[]  DifferentiatorOutMax=[]  FilterDiffOutCoefMin=[]  FilterDiffOutCoefMax=[]  ReciprocalOutMin=[]  ReciprocalOutMax=[]  SumDenOutMin=[]  SumDenOutMax=[]  SumNumOutMin=[]  SumNumOutMax=[]  DivideOutMin=[]  DivideOutMax=[]  UdiffTsProdOutMin=[]  UdiffTsProdOutMax=[]  NTsProdOutMin=[]  NTsProdOutMax=[]  UintegralTsProdOutMin=[]  UintegralTsProdOutMax=[]  UngainTsProdOutMin=[]  UngainTsProdOutMax=[]  ClampingZeroOutDataTypeStr=Inherit: Inherit via back propagation  ClampingZeroOutMin=[]  ClampingZeroOutMax=[]  FilterDenConstantOutDataTypeStr=Inherit: Inherit via back propagation  FilterDenConstantOutMin=[]  FilterDenConstantOutMax=[]  PCopyOutDataTypeStr=Inherit: Inherit via back propagation  PCopyOutMin=[]  PCopyOutMax=[]  NCopyOutDataTypeStr=Inherit: Inherit via back propagation  NCopyOutMin=[]  NCopyOutMax=[]  IntegratorContinuousStateAttributes=''  IntegratorStateMustResolveToSignalObject=off  IntegratorRTWStateStorageClass=Auto  FilterContinuousStateAttributes=''  FilterStateMustResolveToSignalObject=off  FilterRTWStateStorageClass=Auto  ParallelPVariant=InternalParameters  IdealPVariant=Disabled  IVariant=InternalParameters  DVariant=Disabled  IntegratorVariant=Discrete  SatVariant=Enabled  AWVariant=BackCalculation  PCopyVariant=Disabled  TRVariant=Disabled  FdbkBlocksVariant=Forward  IdealPFdbkVariant=Disabled  SatFdbkVariant=Disabled  DerivativeFilterVariant=Disabled  NVariant=Disabled  NCopyVariant=Disabled_SignalSpec  FilterICVariant=Disabled  IntegratorICVariant=InternalICs  ExternalResetVariant=Disabled  TRSumVariant=Passthrough  SumFdbkVariant=Disabled  SumVariant=Sum_PI  TsampFilterVariant=InternalTs  TsampNgainVariant=Passthrough  TsampIntegralVariant=Disabled_SignalSpec  ExternalSaturationOutDataTypeStr=Inherit: Same as second input  DerivativeSourceVariant=Disabled  PreIntVariant=InternalPreInt
  S : Outport
  wires:
  iqgRef/1 -> Sum3/1
  Vd/1 -> Add/1
  idgRef/1 -> Sum1/1
  Mux/1 -> Mux1/1
  [idg] -> Product1/2
  Constant/1 -> Mux1/2
  Inverse Park Transform/1 -> Divide/1, "PWM Generator (Three-phase, Three-level)"/1
  Mux1/1 -> Inverse Park Transform/1
  [iqg] -> Product/2
  omega/1 -> Product2/1, Product/1, [omega]
  [omega] -> Product3/1, Product1/1
  Product/1 -> Gain1/1
  Sum4/1 -> Mux/2
  Product1/1 -> "Gain2 "/1
  Add/1 -> Sum2/1
  idg/1 -> Sum1/2, [idg]
  theta/1 -> Inverse Park Transform/2
  Gain1/1 -> Add/2
  Sum2/1 -> Mux/1
  iqr/1 -> Product2/2
  Product2/1 -> Gain2/1
  Gain2/1 -> Add/3
  idr/1 -> Product3/2
  Product3/1 -> Gain3/1
  "Gain2 "/1 -> Add1/1
  Gain3/1 -> Add1/2
  Add1/1 -> Sum4/2
  Variant Source/1 -> S/1
  Divide/1 -> Gain/1
  "PWM Generator (Three-phase, Three-level)"/1 -> Variant Source/1
  iqg/1 -> [iqg], Sum3/2
  d-axis current PI/1 -> Sum2/2
  Sum1/1 -> d-axis current PI/1
  q-axis current PI/1 -> Sum4/1
  Sum3/1 -> q-axis current PI/1
  Add3/1 -> Gain5/1
  Gain5/1 -> "PWM Generator (Three-phase, Three-level)"/2, Divide/2
  Gain/1 -> Variant Source/2
  Vdcp/1 -> Add3/2
  Constant3/1 -> "PWM Generator (Three-phase, Three-level)"/3
  Vdcn/1 -> Add3/1
  "PWM Generator (Three-phase, Three-level)"/2 -> Terminator/1

== system VoltageSourceConverterHVDCTrans/Control/Sending end and receiving end control/Sending end control/Time mode/Measurements/Clarke ==
  abc : Inport
  0 : Fcn  Expr=u(1) + u(2) + u(3)
  K : Gain  Gain=[2 2 1]/3
  Mux : Mux  Inputs=3
  alpha : Fcn  Expr=(u(1) - u(3))*sqrt(3)/2
  beta : Fcn  Expr=-0.5*u(1) + u(2) -0.5*u(3)
  AlphaBeta0 : Outport
  wires:
  beta/1 -> Mux/2
  Mux/1 -> K/1
  abc/1 -> alpha/1, beta/1, 0/1
  alpha/1 -> Mux/1
  0/1 -> Mux/3
  K/1 -> AlphaBeta0/1

== system VoltageSourceConverterHVDCTrans/Control/Sending end and receiving end control/Sending end control/Time mode/Measurements/Clarke1 ==
  abc : Inport
  0 : Fcn  Expr=u(1) + u(2) + u(3)
  K : Gain  Gain=[2 2 1]/3
  Mux : Mux  Inputs=3
  alpha : Fcn  Expr=(u(1) - u(3))*sqrt(3)/2
  beta : Fcn  Expr=-0.5*u(1) + u(2) -0.5*u(3)
  AlphaBeta0 : Outport
  wires:
  K/1 -> AlphaBeta0/1
  0/1 -> Mux/3
  alpha/1 -> Mux/1
  abc/1 -> 0/1, beta/1, alpha/1
  Mux/1 -> K/1
  beta/1 -> Mux/2

== system VoltageSourceConverterHVDCTrans/Control/Sending end and receiving end control/Sending end control/Time mode/Measurements/PQ Calculation ==
  Vd : Inport
  Id : Inport  Port=2
  Iq : Inport  Port=3
  Gain : Gain  Gain=-1
  Product : Product
  Product4 : Product
  P : Outport
  Q : Outport  Port=2
  wires:
  Vd/1 -> Product4/1, Product/1
  Product/1 -> P/1
  Id/1 -> Product/2
  Iq/1 -> Product4/2
  Product4/1 -> Gain/1
  Gain/1 -> Q/1
